simulink model "MATLABFunctionInStateFlow"  (R2026a)
settings: Solver=VariableStepAuto
StartFcn:
  | learning.simulink.modelCallbacks.startFunction(gcs);
StopFcn:
  | learning.simulink.modelCallbacks.stopFunction(gcs);
model workspace (MAT data in the model file):
  courseObject.course = 'stateflow'
  courseObject.chapter = 9
  courseObject.lesson = 3
  courseObject.section = 1
  courseObject.task = 1
libraries: signalChecks x1, simulink x1
CloseFcn:
  | learning.simulink.cleanupOnlineTraining;learning.simulink.Application.getInstance().dduxLogMatlabEvent("ModelClosed");
Description:
  | TrainingCourseModel
settings Model: Creator=PC  LastModifiedBy=PC

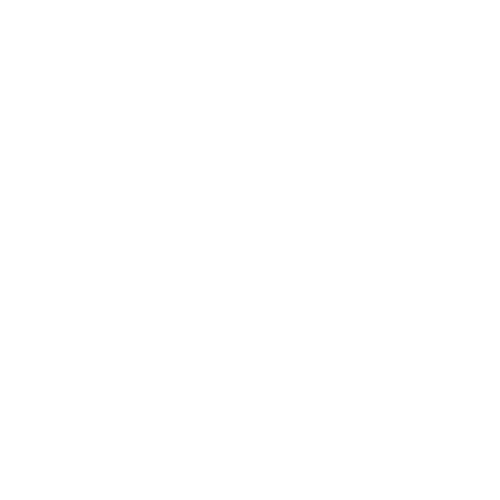
[thumbnail: Simulink's stored preview of the top-level diagram]
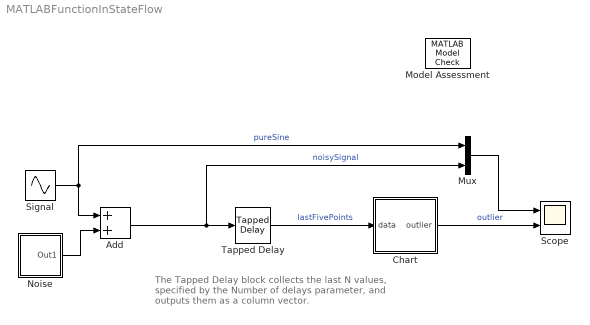
== system MATLABFunctionInStateFlow ==
  note: The Tapped Delay block collects the last N values, specified by the Number of delays parameter, and outputs them as a column vector.
  Add : Sum
  Chart : Stateflow chart  TreatAsAtomicUnit=on
  Model Assessment : signalChecks/MATLAB Model Check  mlfunc='grader_interaction1_task3'  lesson=0  task=3  pass=1
      settings: AttributesFormatString=|
      | No input required
      | for this task
  Mux : Mux  Inputs=2
  Noise : Subsystem
  Scope : Scope  NumInputPorts=2
      settings: ActiveDisplayYMinimum=-5.2454  ActiveDisplayYMaximum=4.59038
  Signal : Sin  SampleTime=0
  Tapped Delay : simulink/Discrete/Tapped Delay  vinit=0.0  samptime=-1  NumDelays=5  DelayOrder=Oldest  includeCurrent=on
  wires:
  Signal/1 -> Add/1, Mux/1  "pureSine"
  Tapped Delay/1 -> Chart/1(data)  "lastFivePoints"
  Add/1 -> Tapped Delay/1, Mux/2  "noisySignal"
  Chart/1(outlier) -> Scope/2  "outlier"
  Noise/1(Out1) -> Add/2
  Mux/1 -> Scope/1

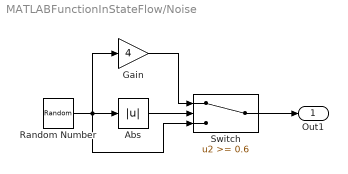
== system MATLABFunctionInStateFlow/Noise ==
  Abs : Abs  SaturateOnIntegerOverflow=off
  Gain : Gain  Gain=4
  Random Number : RandomNumber  Variance=0.1  SampleTime=0.1
  Switch : Switch  Threshold=0.6  SaturateOnIntegerOverflow=off  InputSameDT=off
  Out1 : Outport  VectorParamsAs1DForOutWhenUnconnected=off
  wires:
  Switch/1 -> Out1/1
  Random Number/1 -> Gain/1, Switch/3, Abs/1
  Gain/1 -> Switch/1
  Abs/1 -> Switch/2

== stateflow chart MATLABFunctionInStateFlow/Chart ==
  state NotOutlier
    entry:
    outlier = 0;
  state Outlier
    entry:
    outlier = 1;
  (default) -> NotOutlier
  NotOutlier -> Outlier : [detectOutlier(data)]
  Outlier -> NotOutlier : [~detectOutlier(data)]
  data: input function_input; isOutlier function_output; outlier output; data input
  function isOutlier = detectOutlier(input):
    | function isOutlier = detectOutlier(input)
    | 
    | %Calculate the distance of the last point from the mean
    | dist = abs(input(end) - mean(input));
    | 
    | %Determine if that point was an outlier
    | isOutlier = dist > 2;
